simulink model "single_phase_inverter"  (R2026a)
settings: Solver=ode23tb  StopTime=param.sim.simlength  FixedStep=tc  MaxStep=param.glb_time.tc
values from neighbouring files (symbols this model uses):
  param = add_template_extras(param, options)    [init_model.m]
libraries: fl_lib x45, nesl_utility x24, single_phase_transformer_lib x3, phase_shift_filter x2, phase_shift_filter_ccaller x2, three_phase_voltage_with_frt_emulator x1, power_meter_iec x1, single_phase_transformer x1, three_phase_diode_rectifier x1, three_phase_diode_rectifier_with_thermal_model x1, full_bridge_ideal_switch x1, full_bridge_mosfet_based_with_thermal_model x1
(part 1 of 4)
settings Model: SimulationMode=accelerator  Creator=LTNBDA  LastModifiedBy=d.bagnara
settings SolverCC: ZeroCrossControl=DisableAll  ZeroCrossAlgorithm=Adaptive  SolverResetMethod=Robust
settings DataIOCC: MaxDataPoints=1  SignalLoggingSaveFormat=ModelDataLogs
settings OptimizationCC: InitFltsAndDblsToZero=on  EfficientMapNaN2IntZero=off
settings DebuggingCC: SaveWithParameterizedLinksMsg=none  SignalResolutionControl=TryResolveAllWithWarning  IgnoredZcDiagnostic=none  MultiTaskDSMMsg=warning  MultiTaskCondExecSysMsg=none  MultiTaskRateTransMsg=warning
settings HardwareCC: ProdBitPerLong=64.0  ProdHWDeviceType=Generic->64-bit Embedded Processor (LP64)  TargetBitPerPointer=64.0  TargetBitPerSizeT=64.0  TargetBitPerPtrDiffT=64.0  TargetLongLongMode=on  TargetIntDivRoundTo=Zero  TargetEndianess=LittleEndian  TargetWordSize=64.0  TargetHWDeviceType=MATLAB Host  ProdEqTarget=off
settings SFSimCC: SimCustomHeaderCode=|
  | #include "phase_shift_flt_simulink.h"
  | #include "sv_pwm.h"
  | #include "rpi.h"
  | #include "rpi_simulink.h"
  | #include "first_harmonic_tracker.h"
  | #include "dqvector_pi.h"
  | #include "dqvector_pi_simulink.h"
  | #include "sv_pwm_simulink.h"
  | #include "dqpll_grid.h"
  | #include "first_harmonic_tracker_simulink.h"
  | #include "dqpll_grid_simulink.h"
  | #include "phase_shift_flt.h"
  | #include "math_f.h"
  | #include "linear_double_integrator_observer_simulink.h"
  | #include "linear_double_integrator_observer.h"
  | #include "sogi_flt_simulink.h"
  | #include "sogi_flt.h"
settings SFSimCC: SimUserSources=|
  | "rpi.c"
  | "rpi_simulink.c"
  | "dqvector_pi_simulink.c"
  | "dqvector_pi.c"
  | "sv_pwm_simulink.c"
  | "sv_pwm.c"
  | "first_harmonic_tracker_simulink.c"
  | "first_harmonic_tracker.c"
  | "dqpll_grid_simulink.c"
  | "dqpll_grid.c"
  | "phase_shift_flt_simulink.c"
  | "phase_shift_flt.c"
  | "linear_double_integrator_observer_simulink.c"
  | "linear_double_integrator_observer.c"
  | "sogi_flt_simulink.c"
  | "sogi_flt.c"
settings SFSimCC: SimUserIncludeDirs=|
  | include
  | src
settings CodeAppCC: MaxIdLength=128.0
settings GRTTargetCC: CombineOutputUpdateFcns=off  GRTInterface=on
settings SimscapeCC: SimscapeNormalizeSystem=off  SimscapeNominalValues="[{\"value\":\"1\",\"unit\":\"A\"},{\"value\":\"1\",\"unit\":\"bar\"},{\"value\":\"1\",\"unit\":\"cm^2\"},{\"value\":\"1\",\"unit\":\"cm^3/s\"},{\"value\":\"1\",\"unit\":\"kJ/kg\"},{\"value\":\"1\",\"unit\":\"kW\"},{\"value\":\"1\",\"unit\":\"l\"},{\"value\":\"1\",\"unit\":\"N\"},{\"value\":\"1\",\"unit\":\"N*m\"},{\"value\":\"1\",\"unit\":\"V\"}]"  SimscapeLogType=none  SimscapeLogDataHistory=5000.0

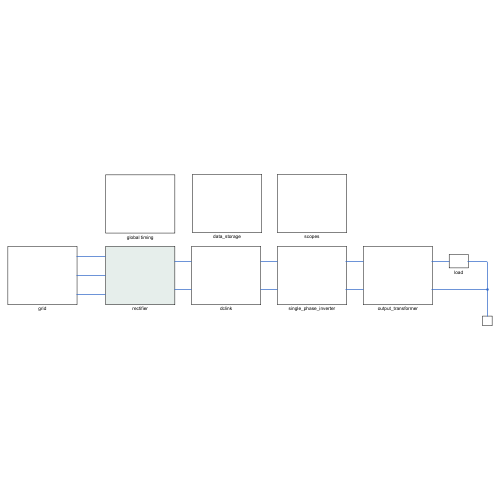
[thumbnail: Simulink's stored preview of the top-level diagram]
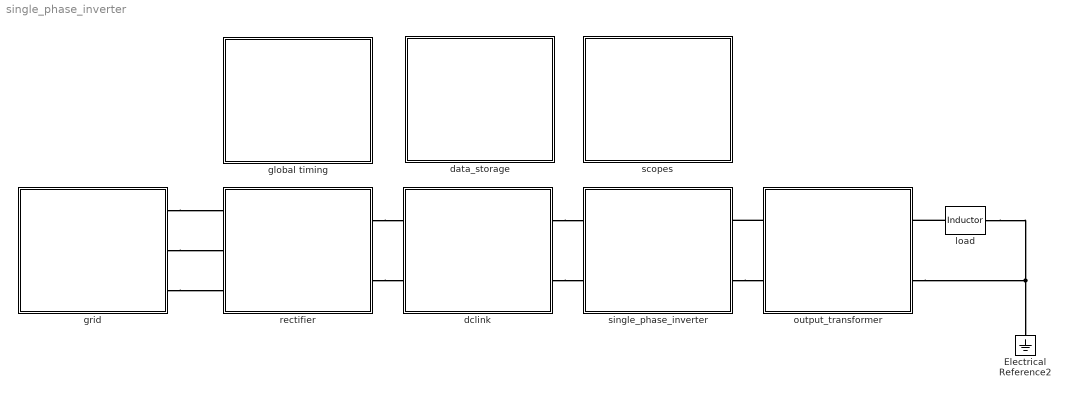
== system single_phase_inverter ==
  Electrical Reference2 : fl_lib/Electrical/Electrical Elements/Electrical Reference
  data_storage : Subsystem
  dclink : Subsystem
  global timing : Subsystem
  grid : Subsystem
  load : fl_lib/Electrical/Electrical Elements/Inductor  l=param.trafo_load.lload H  r=param.trafo_load.rload Ohm  g=1e-9 1/Ohm  i_specify=off  i_priority=None  i=0 A  i_nominal_specify=off  i_nominal_value=1  i_nominal_unit=A  v_specify=off  v_priority=None  v=0 V  v_nominal_specify=off  v_nominal_value=1  v_nominal_unit=V  i_L_specify=off  i_L_priority=High  i_L=0 A  i_L_nominal_specify=off  i_L_nominal_value=1  i_L_nominal_unit=A
  output_transformer : Subsystem
  rectifier : Subsystem
  scopes : Subsystem
  single_phase_inverter : Subsystem
  connections:
  dclink/RConn2 -- single_phase_inverter/LConn2
  dclink/RConn1 -- single_phase_inverter/LConn1
  rectifier/RConn1 -- dclink/LConn1
  rectifier/RConn2 -- dclink/LConn2
  output_transformer/LConn1 -- single_phase_inverter/RConn1
  single_phase_inverter/RConn2 -- output_transformer/LConn2
  output_transformer/RConn2 -- load/RConn1 -- Electrical Reference2/LConn1
  load/LConn1 -- output_transformer/RConn1
  grid/RConn3 -- rectifier/LConn3
  grid/RConn2 -- rectifier/LConn2
  grid/RConn1 -- rectifier/LConn1

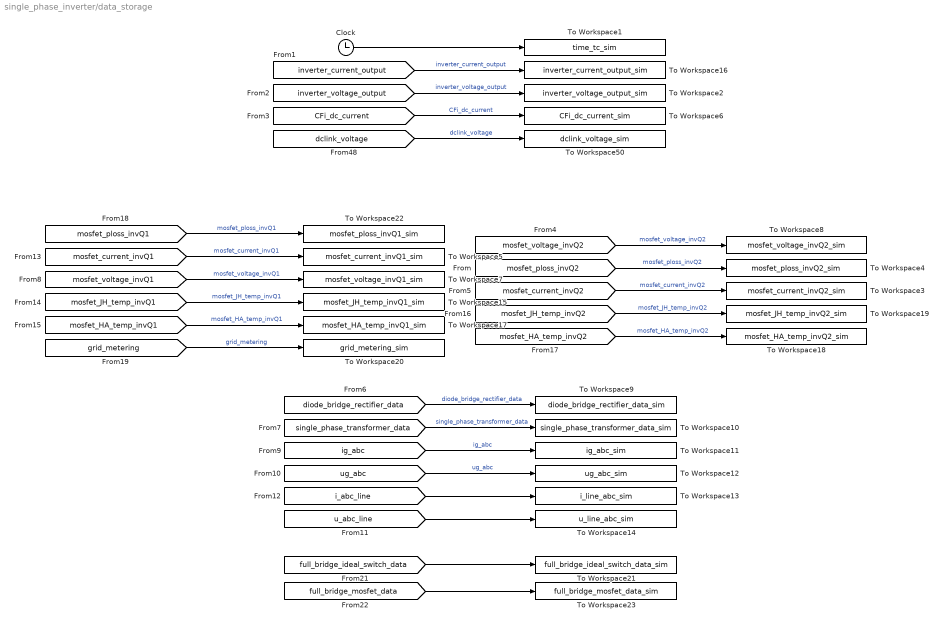
== system single_phase_inverter/data_storage ==
  Clock : Clock
  To Workspace1 : ToWorkspace  VariableName=time_tc_sim  SampleTime=param.glb_time.tc
      settings: MaxDataPoints=param.glb_time.Nc  Decimation=param.glb_time.decimation_tc
  To Workspace10 : ToWorkspace  VariableName=single_phase_transformer_data_sim  SampleTime=param.glb_time.tc
      settings: MaxDataPoints=param.glb_time.Nc  Decimation=param.glb_time.decimation_tc
  To Workspace11 : ToWorkspace  VariableName=ig_abc_sim  SampleTime=param.glb_time.tc
      settings: MaxDataPoints=param.glb_time.Nc  Decimation=param.glb_time.decimation_tc
  To Workspace12 : ToWorkspace  VariableName=ug_abc_sim  SampleTime=param.glb_time.tc
      settings: MaxDataPoints=param.glb_time.Nc  Decimation=param.glb_time.decimation_tc
  To Workspace13 : ToWorkspace  VariableName=i_line_abc_sim  SampleTime=param.glb_time.tc
      settings: MaxDataPoints=param.glb_time.Nc  Decimation=param.glb_time.decimation_tc
  To Workspace14 : ToWorkspace  VariableName=u_line_abc_sim  SampleTime=param.glb_time.tc
      settings: MaxDataPoints=param.glb_time.Nc  Decimation=param.glb_time.decimation_tc
  To Workspace15 : ToWorkspace  VariableName=mosfet_JH_temp_invQ1_sim  SampleTime=param.glb_time.tc
      settings: MaxDataPoints=param.glb_time.Nc  Decimation=param.glb_time.decimation_tc
  To Workspace16 : ToWorkspace  VariableName=inverter_current_output_sim  SampleTime=param.glb_time.tc
      settings: MaxDataPoints=param.glb_time.Nc  Decimation=param.glb_time.decimation_tc
  To Workspace17 : ToWorkspace  VariableName=mosfet_HA_temp_invQ1_sim  SampleTime=param.glb_time.tc
      settings: MaxDataPoints=param.glb_time.Nc  Decimation=param.glb_time.decimation_tc
  To Workspace18 : ToWorkspace  VariableName=mosfet_HA_temp_invQ2_sim  SampleTime=param.glb_time.tc
      settings: MaxDataPoints=param.glb_time.Nc  Decimation=param.glb_time.decimation_tc
  To Workspace19 : ToWorkspace  VariableName=mosfet_JH_temp_invQ2_sim  SampleTime=param.glb_time.tc
      settings: MaxDataPoints=param.glb_time.Nc  Decimation=param.glb_time.decimation_tc
  To Workspace2 : ToWorkspace  VariableName=inverter_voltage_output_sim  SampleTime=param.glb_time.tc
      settings: MaxDataPoints=param.glb_time.Nc  Decimation=param.glb_time.decimation_tc
  To Workspace20 : ToWorkspace  VariableName=grid_metering_sim  SampleTime=param.glb_time.tc
      settings: MaxDataPoints=param.glb_time.Nc  Decimation=param.glb_time.decimation_tc
  To Workspace21 : ToWorkspace  VariableName=full_bridge_ideal_switch_data_sim  SampleTime=param.glb_time.tc
      settings: MaxDataPoints=param.glb_time.Nc  Decimation=param.glb_time.decimation_tc
  To Workspace22 : ToWorkspace  VariableName=mosfet_ploss_invQ1_sim  SampleTime=param.glb_time.tc
      settings: MaxDataPoints=param.glb_time.Nc  Decimation=param.glb_time.decimation_tc
  To Workspace23 : ToWorkspace  VariableName=full_bridge_mosfet_data_sim  SampleTime=param.glb_time.tc
      settings: MaxDataPoints=param.glb_time.Nc  Decimation=param.glb_time.decimation_tc
  To Workspace3 : ToWorkspace  VariableName=mosfet_current_invQ2_sim  SampleTime=param.glb_time.tc
      settings: MaxDataPoints=param.glb_time.Nc  Decimation=param.glb_time.decimation_tc
  To Workspace4 : ToWorkspace  VariableName=mosfet_ploss_invQ2_sim  SampleTime=param.glb_time.tc
      settings: MaxDataPoints=param.glb_time.Nc  Decimation=param.glb_time.decimation_tc
  To Workspace5 : ToWorkspace  VariableName=mosfet_current_invQ1_sim  SampleTime=param.glb_time.tc
      settings: MaxDataPoints=param.glb_time.Nc  Decimation=param.glb_time.decimation_tc
  To Workspace50 : ToWorkspace  VariableName=dclink_voltage_sim  SampleTime=param.glb_time.tc
      settings: MaxDataPoints=param.glb_time.Nc  Decimation=param.glb_time.decimation_tc
  To Workspace6 : ToWorkspace  VariableName=CFi_dc_current_sim  SampleTime=param.glb_time.tc
      settings: MaxDataPoints=param.glb_time.Nc  Decimation=param.glb_time.decimation_tc
  To Workspace7 : ToWorkspace  VariableName=mosfet_voltage_invQ1_sim  SampleTime=param.glb_time.tc
      settings: MaxDataPoints=param.glb_time.Nc  Decimation=param.glb_time.decimation_tc
  To Workspace8 : ToWorkspace  VariableName=mosfet_voltage_invQ2_sim  SampleTime=param.glb_time.tc
      settings: MaxDataPoints=param.glb_time.Nc  Decimation=param.glb_time.decimation_tc
  To Workspace9 : ToWorkspace  VariableName=diode_bridge_rectifier_data_sim  SampleTime=param.glb_time.tc
      settings: MaxDataPoints=param.glb_time.Nc  Decimation=param.glb_time.decimation_tc
  wires:
  Clock/1 -> To Workspace1/1
  [inverter_current_output] -> To Workspace16/1  "inverter_current_output"
  [inverter_voltage_output] -> To Workspace2/1  "inverter_voltage_output"
  [CFi_dc_current] -> To Workspace6/1  "CFi_dc_current"
  [mosfet_ploss_invQ1] -> To Workspace22/1  "mosfet_ploss_invQ1"
  [dclink_voltage] -> To Workspace50/1  "dclink_voltage"
  [mosfet_current_invQ1] -> To Workspace5/1  "mosfet_current_invQ1"
  [mosfet_current_invQ2] -> To Workspace3/1  "mosfet_current_invQ2"
  [mosfet_ploss_invQ2] -> To Workspace4/1  "mosfet_ploss_invQ2"
  [mosfet_voltage_invQ1] -> To Workspace7/1  "mosfet_voltage_invQ1"
  [mosfet_voltage_invQ2] -> To Workspace8/1  "mosfet_voltage_invQ2"
  [diode_bridge_rectifier_data] -> To Workspace9/1  "diode_bridge_rectifier_data"
  [single_phase_transformer_data] -> To Workspace10/1  "single_phase_transformer_data"
  [ig_abc] -> To Workspace11/1  "ig_abc"
  [ug_abc] -> To Workspace12/1  "ug_abc"
  [i_abc_line] -> To Workspace13/1
  [u_abc_line] -> To Workspace14/1
  [mosfet_JH_temp_invQ1] -> To Workspace15/1  "mosfet_JH_temp_invQ1"
  [mosfet_HA_temp_invQ1] -> To Workspace17/1  "mosfet_HA_temp_invQ1"
  [mosfet_JH_temp_invQ2] -> To Workspace19/1  "mosfet_JH_temp_invQ2"
  [mosfet_HA_temp_invQ2] -> To Workspace18/1  "mosfet_HA_temp_invQ2"
  [grid_metering] -> To Workspace20/1  "grid_metering"
  [full_bridge_mosfet_data] -> To Workspace23/1
  [full_bridge_ideal_switch_data] -> To Workspace21/1

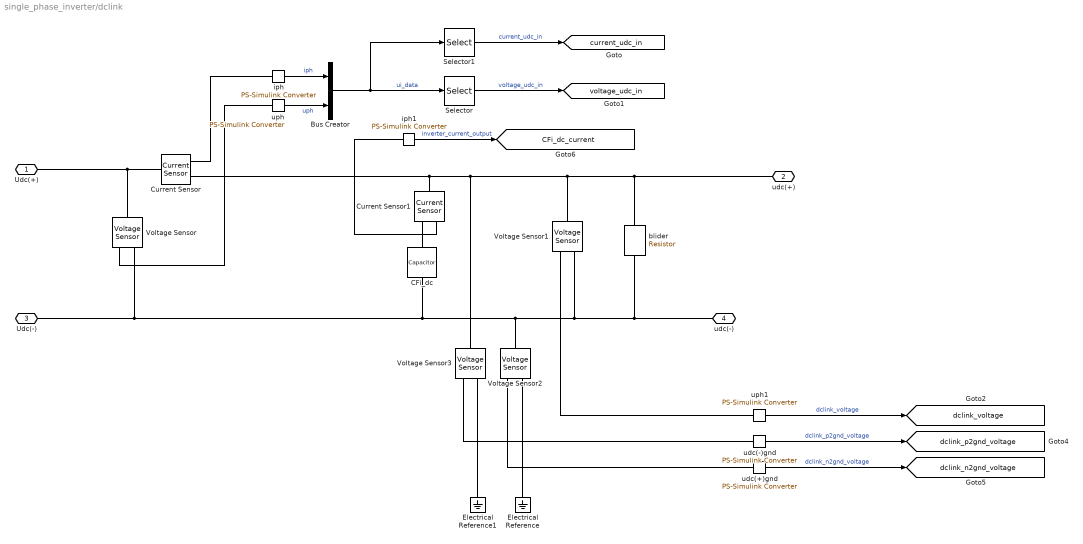
== system single_phase_inverter/dclink ==
  Bus Creator : BusCreator  Inputs=2
  CFi_dc : fl_lib/Electrical/Electrical Elements/Capacitor  c=param.spinv.hw.CFi F  r=param.spinv.hw.RCFi Ohm  g=0 1/Ohm  i_specify=off  i_priority=None  i=0 A  i_nominal_specify=off  i_nominal_value=1  i_nominal_unit=A  v_specify=off  v_priority=None  v=0 V  v_nominal_specify=off  v_nominal_value=1  v_nominal_unit=V  vc_specify=off  vc_priority=High  vc=0 V  vc_nominal_specify=off  vc_nominal_value=1  vc_nominal_unit=V
  Current Sensor : fl_lib/Electrical/Electrical Sensors/Current Sensor
  Current Sensor1 : fl_lib/Electrical/Electrical Sensors/Current Sensor
  Electrical Reference : fl_lib/Electrical/Electrical Elements/Electrical Reference
  Electrical Reference1 : fl_lib/Electrical/Electrical Elements/Electrical Reference
  Selector : Selector  InputPortWidth=2  IndexOptions=Index vector (dialog)  Indices=2  OutputSizes=1
  Selector1 : Selector  InputPortWidth=2  IndexOptions=Index vector (dialog)  Indices=1  OutputSizes=1
  Voltage Sensor{,1..3} (4 alike) : fl_lib/Electrical/Electrical Sensors/Voltage Sensor
  blider : fl_lib/Electrical/Electrical Elements/Resistor  R=1200 Ohm  i_specify=off  i_priority=None  i=0 A  i_nominal_specify=off  i_nominal_value=1  i_nominal_unit=A  v_specify=off  v_priority=None  v=0 V  v_nominal_specify=off  v_nominal_value=1  v_nominal_unit=V
  iph : nesl_utility/PS-Simulink Converter  PhysicalDomain=network_engine_domain  SubClassName=ps_output  LeftPortType=input  RightPortType=output  PseudoPeriodic=off  Frequencies=[]  VectorFormat=1-D array  Unit=A  AffineConversion=off
  iph1 : nesl_utility/PS-Simulink Converter  PhysicalDomain=network_engine_domain  SubClassName=ps_output  LeftPortType=input  RightPortType=output  PseudoPeriodic=off  Frequencies=[]  VectorFormat=1-D array  Unit=A  AffineConversion=off
  udc(+)gnd : nesl_utility/PS-Simulink Converter  PhysicalDomain=network_engine_domain  SubClassName=ps_output  LeftPortType=input  RightPortType=output  PseudoPeriodic=off  Frequencies=[]  VectorFormat=1-D array  Unit=V  AffineConversion=off
  udc(-)gnd : nesl_utility/PS-Simulink Converter  PhysicalDomain=network_engine_domain  SubClassName=ps_output  LeftPortType=input  RightPortType=output  PseudoPeriodic=off  Frequencies=[]  VectorFormat=1-D array  Unit=V  AffineConversion=off
  uph : nesl_utility/PS-Simulink Converter  PhysicalDomain=network_engine_domain  SubClassName=ps_output  LeftPortType=input  RightPortType=output  PseudoPeriodic=off  Frequencies=[]  VectorFormat=1-D array  Unit=V  AffineConversion=off
  uph1 : nesl_utility/PS-Simulink Converter  PhysicalDomain=network_engine_domain  SubClassName=ps_output  LeftPortType=input  RightPortType=output  PseudoPeriodic=off  Frequencies=[]  VectorFormat=1-D array  Unit=V  AffineConversion=off
  Udc(+) : PMIOPort  Side=Left
  udc(+) : PMIOPort  Port=2  Side=Right
  Udc(-) : PMIOPort  Port=3  Side=Left
  udc(-) : PMIOPort  Port=4  Side=Right
  tag scope: CFi_dc_current=global, current_udc_in=global, dclink_n2gnd_voltage=global, dclink_p2gnd_voltage=global, dclink_voltage=global, voltage_udc_in=global
  wires:
  Bus Creator/1 -> Selector/1, Selector1/1  "ui_data"
  iph/1 -> Bus Creator/1  "iph"
  uph/1 -> Bus Creator/2  "uph"
  Selector1/1 -> [current_udc_in]  "current_udc_in"
  Selector/1 -> [voltage_udc_in]  "voltage_udc_in"
  iph1/1 -> [CFi_dc_current]  "inverter_current_output"
  udc(+)gnd/1 -> [dclink_n2gnd_voltage]  "dclink_n2gnd_voltage"
  uph1/1 -> [dclink_voltage]  "dclink_voltage"
  udc(-)gnd/1 -> [dclink_p2gnd_voltage]  "dclink_p2gnd_voltage"
  connections:
  iph/LConn1 -- Current Sensor/RConn1
  Voltage Sensor/LConn1 -- Current Sensor/LConn1 -- Udc(+)/RConn1
  Voltage Sensor/RConn1 -- uph/LConn1
  CFi_dc/RConn1 -- Voltage Sensor1/RConn2 -- udc(-)/RConn1 -- blider/RConn1 -- Voltage Sensor2/LConn1 -- Voltage Sensor/RConn2 -- Udc(-)/RConn1
  udc(+)/RConn1 -- blider/LConn1 -- Voltage Sensor1/LConn1 -- Voltage Sensor3/LConn1 -- Current Sensor/RConn2 -- Current Sensor1/LConn1
  Current Sensor1/RConn2 -- CFi_dc/LConn1
  Electrical Reference1/LConn1 -- Voltage Sensor3/RConn2
  udc(-)gnd/LConn1 -- Voltage Sensor3/RConn1
  Voltage Sensor2/RConn1 -- udc(+)gnd/LConn1
  Electrical Reference/LConn1 -- Voltage Sensor2/RConn2
  Voltage Sensor1/RConn1 -- uph1/LConn1
  Current Sensor1/RConn1 -- iph1/LConn1

== system single_phase_inverter/global timing ==
  Unit Delay : UnitDelay  SampleTime=param.glb_time.tc
  time_afe1 : Subsystem  mask{k=1}
      mask prompts: k "Time Gain"
      mask Display:
      | disp('time-gen');
      | port_label('input', 1, 'crt');
      | port_label('output', 1, 'tout');
  time_afe3 : Subsystem  mask{k=1}
      mask prompts: k "Time Gain"
      mask Display:
      | disp('time-gen');
      | port_label('output', 1, 'tout');
  tag scope: master_time=global, time_inv_module_1=global
  wires:
  time_afe1/1(Out1) -> [time_inv_module_1]
  time_afe3/1(Out1) -> [master_time]
  [local_time_corr_llc_mod1] -> Unit Delay/1
  Unit Delay/1 -> time_afe1/1(correction_time)

== system single_phase_inverter/grid ==
  Bus Selector : BusSelector  OutputSignals=Q1p,Q1n,P1n,P1p,U1n,U1p,i_act_1n,i_react_1n,i_act_1p,i_react_1p
  To Workspace1 : ToWorkspace  VariableName=i_react_1n  SampleTime=param.glb_time.ts_afe
      settings: MaxDataPoints=param.glb_time.Ns_afe
  To Workspace2 : ToWorkspace  VariableName=i_react_1p  SampleTime=param.glb_time.ts_afe
      settings: MaxDataPoints=param.glb_time.Ns_afe
  To Workspace3 : ToWorkspace  VariableName=i_act_1n  SampleTime=param.glb_time.ts_afe
      settings: MaxDataPoints=param.glb_time.Ns_afe
  To Workspace4 : ToWorkspace  VariableName=i_act_1p  SampleTime=param.glb_time.ts_afe
      settings: MaxDataPoints=param.glb_time.Ns_afe
  To Workspace5 : ToWorkspace  VariableName=u1p  SampleTime=param.glb_time.ts_afe
      settings: MaxDataPoints=param.glb_time.Ns_afe
  To Workspace6 : ToWorkspace  VariableName=u1n  SampleTime=param.glb_time.ts_afe
      settings: MaxDataPoints=param.glb_time.Ns_afe
  grid_emulator : Subsystem
  power meter iec : power_meter_iec/power meter iec  period=pi/param.grid.emu.omega_grid_nom  ts=param.glb_time.ts_afe  enable_time=0.025
  threephase_vi_measures : Subsystem
  ua : PMIOPort  Side=Right
  ub : PMIOPort  Port=2  Side=Right
  uc : PMIOPort  Port=3  Side=Right
  tag scope: P1n_global=global, P1p_global=global, Q1n_global=global, Q1p_global=global, grid_metering=global
  wires:
  [gamma_grid_emulator] -> power meter iec/1
  [ug_abc] -> power meter iec/2
  [ig_abc] -> power meter iec/3
  power meter iec/1 -> [grid_metering], Bus Selector/1
  Bus Selector/1 -> [Q1p_global]  "<Q1p>"
  Bus Selector/2 -> [Q1n_global]  "<Q1n>"
  Bus Selector/3 -> [P1n_global]  "<P1n>"
  Bus Selector/4 -> [P1p_global]  "<P1p>"
  Bus Selector/5 -> To Workspace6/1  "<U1n>"
  Bus Selector/6 -> To Workspace5/1  "<U1p>"
  Bus Selector/7 -> To Workspace3/1  "<i_act_1n>"
  Bus Selector/8 -> To Workspace1/1  "<i_react_1n>"
  Bus Selector/9 -> To Workspace4/1  "<i_act_1p>"
  Bus Selector/10 -> To Workspace2/1  "<i_react_1p>"
  [omega_grid_emulator] -> power meter iec/4
  connections:
  threephase_vi_measures/LConn3 -- grid_emulator/RConn3
  threephase_vi_measures/LConn1 -- grid_emulator/RConn1
  threephase_vi_measures/RConn2 -- ub/RConn1
  threephase_vi_measures/LConn2 -- grid_emulator/RConn2
  threephase_vi_measures/RConn1 -- ua/RConn1
  threephase_vi_measures/RConn3 -- uc/RConn1

== system single_phase_inverter/output_transformer ==
  single_phase_transformer : single_phase_transformer/single_phase_transformer  lm_trafo=param.trafo_load.output_transformer.Lm1  m1=param.trafo_load.output_transformer.n1  m2=param.trafo_load.output_transformer.n2  rd1_trafo=param.trafo_load.output_transformer.Rd1  rd2_trafo=0  ld1_trafo=2*param.trafo_load.output_transformer.Ld1  ld2_trafo=0  rfe_trafo=param.trafo_load.output_transformer.Rfe1  length_core=1  mu0=1.256637e-6  mur=1200
  single_phase_transformer - scope : Scope
      settings: ActiveDisplayYMinimum=-52667.127888169394  ActiveDisplayYMaximum=52594.361496045676  DataLoggingVariableName=ScopeData11
  u1(+) : PMIOPort  Side=Left
  u2(+) : PMIOPort  Port=2  Side=Right
  u1(-) : PMIOPort  Port=3  Side=Left
  u2(-) : PMIOPort  Port=4  Side=Right
  tag scope: single_phase_transformer_data=global
  wires:
  single_phase_transformer/1 -> [single_phase_transformer_data], single_phase_transformer - scope/1
  connections:
  single_phase_transformer/LConn2 -- u1(-)/RConn1
  single_phase_transformer/LConn1 -- u1(+)/RConn1
  single_phase_transformer/RConn1 -- u2(+)/RConn1
  single_phase_transformer/RConn2 -- u2(-)/RConn1

== system single_phase_inverter/rectifier ==
  H5_filter : Subsystem  Commented=on
  H7_filter : Subsystem  Commented=on
  three phase diode rectifier : three_phase_diode_rectifier/three phase diode rectifier  Commented=on  Vf_diode_rectifier=param.diode.rectifier.Vf  Rdon_diode_rectifier=param.diode.rectifier.Rdon  Csnubber=param.spinv.igbt.Csnubber  Rsnubber=param.spinv.igbt.Rsnubber
  three_phase_diode_rectifier_with_thermal_model : three_phase_diode_rectifier_with_thermal_model/three_phase_diode_rectifier_with_thermal_model  Vf_diode_rectifier=param.diode.rectifier.Vf  Rdon_diode_rectifier=param.diode.rectifier.Rdon  mass_heatsink_m=param.thermal.heatsink.no_weight  specific_heat_m=param.thermal.heatsink.cp  rth_diode_JH_m=param.spinv.igbt.Rth_diode_JH  rth_diode_HA_m=param.thermal.Rth_mosfet_HA  Csnubber=param.spinv.igbt.Csnubber  Rsnubber=param.spinv.igbt.Rsnubber
      link override diode_3/Goto2: GotoTag=diode3_JH_temperature
  us_a : PMIOPort  Side=Left
  us_b : PMIOPort  Port=2  Side=Left
  us_c : PMIOPort  Port=3  Side=Left
  Udc(+) : PMIOPort  Port=4  Side=Right
  Udc(-) : PMIOPort  Port=5  Side=Right
  tag scope: diode_bridge_rectifier_data=global
  wires:
  three_phase_diode_rectifier_with_thermal_model/1 -> [diode_bridge_rectifier_data]
  connections:
  Udc(+)/RConn1 -- three_phase_diode_rectifier_with_thermal_model/RConn1 -- three phase diode rectifier/RConn1
  Udc(-)/RConn1 -- three_phase_diode_rectifier_with_thermal_model/RConn2 -- three phase diode rectifier/RConn2
  H5_filter/LConn1 -- us_a/RConn1 -- three_phase_diode_rectifier_with_thermal_model/LConn1 -- three phase diode rectifier/LConn1 -- H7_filter/LConn1
  H5_filter/LConn2 -- us_b/RConn1 -- three phase diode rectifier/LConn2 -- three_phase_diode_rectifier_with_thermal_model/LConn2 -- H7_filter/LConn2
  H5_filter/LConn3 -- us_c/RConn1 -- three_phase_diode_rectifier_with_thermal_model/LConn3 -- three phase diode rectifier/LConn3 -- H7_filter/LConn3

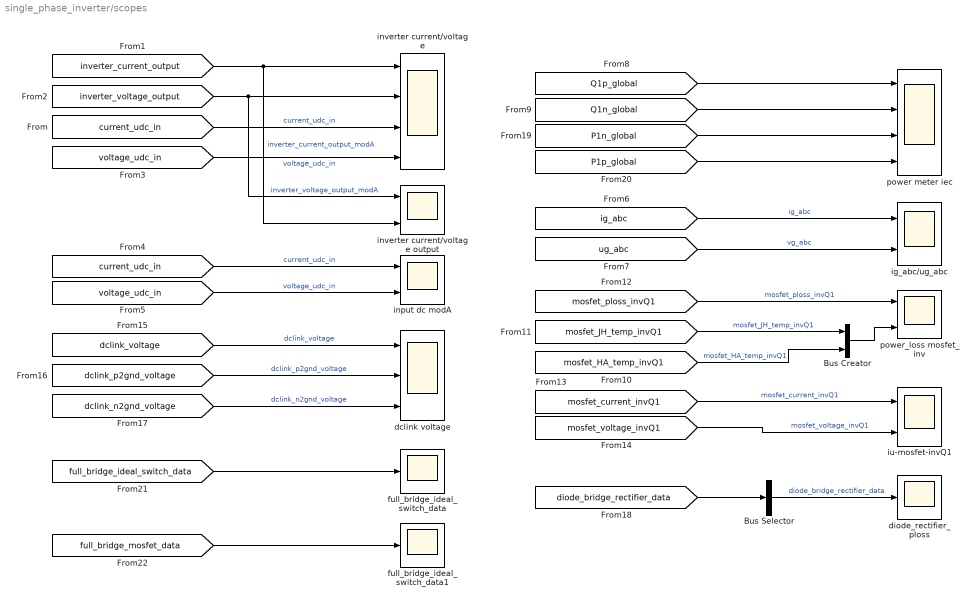
== system single_phase_inverter/scopes ==
  Bus Creator : BusCreator  Inputs=2
  Bus Selector : BusSelector  OutputSignals=diode1_ploss,diode6_ploss,diode5_ploss,diode4_ploss,diode3_ploss,diode2_ploss  OutputAsBus=on
  dclink voltage : Scope  NumInputPorts=3
      settings: SampleTime=param.glb_time.tc  ActiveDisplayString=3  ActiveDisplayYMinimum=-363.18697781386322  ActiveDisplayYMaximum=-188.17161920145585  DataLoggingVariableName=ScopeData9
  diode_rectifier_ploss : Scope
      settings: ActiveDisplayYMinimum=-388.41488046396341  ActiveDisplayYMaximum=3494.091610714474  DataLoggingVariableName=ScopeData13
  full_bridge_ideal_switch_data : Scope
      settings: ActiveDisplayYMinimum=-388.41488046396341  ActiveDisplayYMaximum=3494.091610714474  DataLoggingVariableName=ScopeData17
  full_bridge_ideal_switch_data1 : Scope
      settings: ActiveDisplayYMinimum=-388.41488046396341  ActiveDisplayYMaximum=3494.091610714474  DataLoggingVariableName=ScopeData18
  ig_abc/ug_abc : Scope  NumInputPorts=2
      settings: SampleTime=param.glb_time.tc  ActiveDisplayYMinimum=-781.78189031693421  ActiveDisplayYMaximum=781.86071704862093  DataLoggingVariableName=ScopeData5
  input dc modA : Scope  NumInputPorts=2
      settings: SampleTime=param.glb_time.tc  ActiveDisplayYMinimum=-264.41735822415785  ActiveDisplayYMaximum=1802.2815575209611  DataLoggingVariableName=ScopeData4
  inverter current/voltage : Scope  NumInputPorts=4
      settings: ActiveDisplayString=3  ActiveDisplayYMinimum=-93.6274374097306  ActiveDisplayYMaximum=842.6107714271742
  inverter current/voltage output : Scope  NumInputPorts=2
      settings: ActiveDisplayYMinimum=-719.5057944888872  ActiveDisplayYMaximum=719.52818794442339
  iu-mosfet-invQ1 : Scope  NumInputPorts=2
      settings: SampleTime=param.glb_time.tc  ActiveDisplayYMinimum=-1884.5917198054758  ActiveDisplayYMaximum=2532.7760155502147  DataLoggingVariableName=ScopeData7
  power meter iec : Scope  NumInputPorts=4
      settings: ActiveDisplayString=3  ActiveDisplayYMinimum=-178.52926094214885  ActiveDisplayYMaximum=1606.7629741781627  DataLoggingVariableName=ScopeData16
  power_loss mosfet_inv : Scope  NumInputPorts=2
      settings: SampleTime=param.glb_time.tc  ActiveDisplayYMinimum=-70.3597503046535  ActiveDisplayYMaximum=633.23512274412  DataLoggingVariableName=ScopeData6
  wires:
  [current_udc_in] -> inverter current/voltage/3  "current_udc_in"
  [inverter_voltage_output] -> inverter current/voltage output/1, inverter current/voltage/2  "inverter_voltage_output_modA"
  [inverter_current_output] -> inverter current/voltage output/2, inverter current/voltage/1  "inverter_current_output_modA"
  [voltage_udc_in] -> inverter current/voltage/4  "voltage_udc_in"
  [current_udc_in] -> input dc modA/1  "current_udc_in"
  [voltage_udc_in] -> input dc modA/2  "voltage_udc_in"
  [ug_abc] -> ig_abc/ug_abc/2  "vg_abc"
  [ig_abc] -> ig_abc/ug_abc/1  "ig_abc"
  [mosfet_ploss_invQ1] -> power_loss mosfet_inv/1  "mosfet_ploss_invQ1"
  [mosfet_JH_temp_invQ1] -> Bus Creator/1  "mosfet_JH_temp_invQ1"
  [mosfet_HA_temp_invQ1] -> Bus Creator/2  "mosfet_HA_temp_invQ1"
  Bus Creator/1 -> power_loss mosfet_inv/2
  [mosfet_current_invQ1] -> iu-mosfet-invQ1/1  "mosfet_current_invQ1"
  [mosfet_voltage_invQ1] -> iu-mosfet-invQ1/2  "mosfet_voltage_invQ1"
  [dclink_voltage] -> dclink voltage/1  "dclink_voltage"
  [dclink_p2gnd_voltage] -> dclink voltage/2  "dclink_p2gnd_voltage"
  [dclink_n2gnd_voltage] -> dclink voltage/3  "dclink_n2gnd_voltage"
  [diode_bridge_rectifier_data] -> Bus Selector/1
  Bus Selector/1 -> diode_rectifier_ploss/1  "diode_bridge_rectifier_data"
  [Q1p_global] -> power meter iec/1
  [Q1n_global] -> power meter iec/2
  [P1n_global] -> power meter iec/3
  [P1p_global] -> power meter iec/4
  [full_bridge_ideal_switch_data] -> full_bridge_ideal_switch_data/1
  [full_bridge_mosfet_data] -> full_bridge_ideal_switch_data1/1

== system single_phase_inverter/single_phase_inverter ==
  Current Sensor : fl_lib/Electrical/Electrical Sensors/Current Sensor
  Voltage Sensor1 : fl_lib/Electrical/Electrical Sensors/Voltage Sensor
  iph : nesl_utility/PS-Simulink Converter  PhysicalDomain=network_engine_domain  SubClassName=ps_output  LeftPortType=input  RightPortType=output  PseudoPeriodic=off  Frequencies=[]  VectorFormat=1-D array  Unit=A  AffineConversion=off
  single phase inverter : Subsystem
      settings: PortSchema="{\"entries\":[{\"content\":{\"sides\":[{\"content\":{\"connectorIds\":[\"LConn1\",\"LConn2\"]},\"type\":\"ConnectorPlacement.EquallySpacedRectSide\",\"uuid\":\"4fcf4fea-d38f-431b-8a91-be3ce9782faf\"},{\"content\":{\"connectorIds\":[\"RConn1\",\"RConn2\"],\"side\":\"RIGHT\"},\"type\":\"ConnectorPlacement.EquallySpacedRectSide\",\"uuid\":\"0aa56277-92e9-4e3b-84c7-43398254a4d8\"},{\"content\":{\"connectorIds\":[\"In1\"],\"side\":\"TOP\"},\"type\":\"ConnectorPlacement.EquallySpacedRectSide\",\"uuid\":\"5cd150dc-bcaf-4cd7-b2a8-3db203726730\"}]},\"type\":\"ConnectorPlacement.EquallySpacedConnector\",\"uuid\":\"bf8194c4-c327-4d40-bea4-f1e7617f80b4\"}],\"packageUris\":[\"http://schema.mathworks.com/mf0/Connector/R2020b\"],\"version\":\"1.0\"}"
  single phase inverter control : Subsystem
  uph1 : nesl_utility/PS-Simulink Converter  PhysicalDomain=network_engine_domain  SubClassName=ps_output  LeftPortType=input  RightPortType=output  PseudoPeriodic=off  Frequencies=[]  VectorFormat=1-D array  Unit=V  AffineConversion=off
  uac(+) : PMIOPort  Side=Right
  uac(-) : PMIOPort  Port=2  Side=Right
  udc(+) : PMIOPort  Port=3  Side=Left
  udc(-) : PMIOPort  Port=4  Side=Left
  tag scope: inverter_current_output=global, inverter_voltage_output=global
  wires:
  single phase inverter control/1(gate_cmds) -> single phase inverter/1(gate_commands)
  iph/1 -> [inverter_current_output]  "inverter_current_output"
  uph1/1 -> [inverter_voltage_output]  "inverter_voltage_output"
  connections:
  Current Sensor/LConn1 -- single phase inverter/LConn1
  uac(-)/RConn1 -- single phase inverter/LConn2 -- Voltage Sensor1/RConn2
  Voltage Sensor1/RConn1 -- uph1/LConn1
  iph/LConn1 -- Current Sensor/RConn1
  uac(+)/RConn1 -- Current Sensor/RConn2 -- Voltage Sensor1/LConn1
  udc(+)/RConn1 -- single phase inverter/RConn1
  udc(-)/RConn1 -- single phase inverter/RConn2

== system single_phase_inverter/global timing/time_afe1 ==
  correction_time : Inport
  Constant : Constant
  Gain : Gain  Gain=k
  Product : Product
  Sum : Sum  Inputs=|++
  time_1 : Clock
  Out1 : Outport
  wires:
  time_1/1 -> Gain/1
  Gain/1 -> Product/1
  Product/1 -> Out1/1
  correction_time/1 -> Sum/1
  Sum/1 -> Product/2
  Constant/1 -> Sum/2

== system single_phase_inverter/global timing/time_afe3 ==
  Gain : Gain  Gain=k
  time_1 : Clock
  Out1 : Outport
  wires:
  Gain/1 -> Out1/1
  time_1/1 -> Gain/1

== system single_phase_inverter/grid/grid_emulator ==
  3ph_Dyg : Subsystem
  Bus Selector : BusSelector  OutputSignals=ua_grid_emu,ub_grid_emu,uc_grid_emu
  Bus Selector1 : BusSelector  OutputSignals=gamma_grid_emulator,omega_grid_emulator
  Controlled Voltage Source : fl_lib/Electrical/Electrical Sources/Controlled Voltage Source
  Controlled Voltage Source1 : fl_lib/Electrical/Electrical Sources/Controlled Voltage Source
  Controlled Voltage Source2 : fl_lib/Electrical/Electrical Sources/Controlled Voltage Source
  Electrical Reference : fl_lib/Electrical/Electrical Elements/Electrical Reference
  Simulink-PS Converter : nesl_utility/Simulink-PS Converter  PhysicalDomain=network_engine_domain  SubClassName=ps_input  LeftPortType=input  RightPortType=output  PseudoPeriodic=off  Frequencies=[]  NoiseDistribution=none  NoiseParameters=[]  Unit=V  AffineConversion=on  FilteringAndDerivatives=provide  SimscapeFilterOrder=1  InputFilterTimeConstant=0.001  UdotUserProvided=0
  Simulink-PS Converter1 : nesl_utility/Simulink-PS Converter  PhysicalDomain=network_engine_domain  SubClassName=ps_input  LeftPortType=input  RightPortType=output  PseudoPeriodic=off  Frequencies=[]  NoiseDistribution=none  NoiseParameters=[]  Unit=V  AffineConversion=on  FilteringAndDerivatives=provide  SimscapeFilterOrder=1  InputFilterTimeConstant=0.001  UdotUserProvided=0
  Simulink-PS Converter2 : nesl_utility/Simulink-PS Converter  PhysicalDomain=network_engine_domain  SubClassName=ps_input  LeftPortType=input  RightPortType=output  PseudoPeriodic=off  Frequencies=[]  NoiseDistribution=none  NoiseParameters=[]  Unit=V  AffineConversion=on  FilteringAndDerivatives=provide  SimscapeFilterOrder=1  InputFilterTimeConstant=0.001  UdotUserProvided=0
  Solver Configuration : nesl_utility/Solver Configuration  PhysicalDomain=network_engine_domain  SubClassName=solver  LeftPortType=input  RightPortType=generic  Tones=[]  Harmonics=[]  SimulateNoise=off  Profile=off  UseLocalSampling=off  EnableSwitchedLinearOptims=on  FrequencyDomain=off  UseCCode=off  RelTol=0.001  AbsTol=0.001  MinStep=1e-09  ToWorkspace=off  RevertToSquareIcSolve=off  NumHomotopyIterations=100  PhasorMode=off  PhasorModeNumHarmonics=1  ConsistencySolver=NEWTON_FTOL  CanonicalOrdering=UNORDERED  OptimizeIntermediates=UNOPTIMIZED  IndexReductionMethod=DerivativeReplacement  DoDC=on  ResidualTolerance=1e-09  ConsistencyTolSource=GLOBAL  ConsistencyAbsTol=0.001  ConsistencyRelTol=0.001  ConsistencyTolFactor=0.001  UseLocalSolver=on  LocalSolverChoice=NE_BACKWARD_EULER_ADVANCER  ResolveIndetEquations=on  FunctionEvalNumThread=1  LocalSolverSampleTime=param.glb_time.tc  DoFixedCost=on  MaxNonlinIter=param.sim.nonlinear_iterations  MaxModeIter=2  ComputeImpulses=off  ImpulseIterations=2  LinearAlgebra=auto  LinearAlgebraNumThread=0  EquationFormulation=NE_TIME_EF  DelaysMemoryBudget=1024  AutomaticFiltering=on  FilteringTimeConstant=0.001  PartitionStorageMethod=AS_NEEDED  PartitionMemoryBudget=1024  PartitionMethod=ROBUST  MultibodyUseLocalSolver=off  MultibodyLocalSolverChoice=ODE1  MultibodyLocalSolverSampleTime=0.001
  three_phase_voltage_source_with_frt_emulator : three_phase_voltage_with_frt_emulator/three_phase_voltage_source_with_frt_emulator  nominal_frequency_m=param.grid.emu.fgrid_nom  nominal_voltage_m=param.grid.emu.us_primary_nom  Vemu_ref_norm_m=param.grid.emu.Vemu_ref_norm  vp_xi_pu_m=param.grid.emu.up_xi_pu_ref  vp_eta_pu_m=param.grid.emu.up_eta_pu_ref  vn_xi_pu_m=param.grid.emu.un_xi_pu_ref  vn_eta_pu_m=param.grid.emu.un_eta_pu_ref  Am=param.ctrl.filters.afe.SOF_50Hz.ss_c.A  Bm=param.ctrl.filters.afe.SOF_50Hz.ss_c.B  Cm=param.ctrl.filters.afe.SOF_50Hz.ss_c.C  enable_frt_1_m=param.frt.data.enable_frt_1  enable_frt_2_m=param.frt.data.enable_frt_2  start_time_LVRT_m=param.frt.data.start_time_LVRT  end_time_LVRT_m=param.frt.data.end_time_LVRT  deepPOSxi_m=param.frt.data.deepPOSxi  deepPOSeta_m=param.frt.data.deepPOSeta  deepNEGxi_m=param.frt.data.deepNEGxi  deepNEGeta_m=param.frt.data.deepNEGeta  Amplitude_U_m=param.frt.data.Amplitude_U  Amplitude_V_m=param.frt.data.Amplitude_V  Amplitude_W_m=param.frt.data.Amplitude_W  t_ramp_m=param.frt.data.t_ramp  Phase_shift_m=param.frt.data.Phase_shift
  threephase_vi_measures : Subsystem
  u1 : PMIOPort  Side=Right
  u2 : PMIOPort  Port=2  Side=Right
  u3 : PMIOPort  Port=3  Side=Right
  tag scope: gamma_grid_emulator=global, omega_grid_emulator=global
  wires:
  Bus Selector1/2 -> [omega_grid_emulator]  "<omega_grid_emulator>"
  Bus Selector1/1 -> [gamma_grid_emulator]  "<gamma_grid_emulator>"
  Bus Selector/2 -> Simulink-PS Converter1/1  "<ub_grid_emu>"
  Bus Selector/3 -> Simulink-PS Converter2/1  "<uc_grid_emu>"
  three_phase_voltage_source_with_frt_emulator/1 -> Bus Selector1/1, Bus Selector/1
  Bus Selector/1 -> Simulink-PS Converter/1  "<ua_grid_emu>"
  connections:
  Simulink-PS Converter/RConn1 -- Controlled Voltage Source/RConn1
  Simulink-PS Converter1/RConn1 -- Controlled Voltage Source1/RConn1
  Simulink-PS Converter2/RConn1 -- Controlled Voltage Source2/RConn1
  Controlled Voltage Source/RConn2 -- Controlled Voltage Source1/RConn2 -- Controlled Voltage Source2/RConn2 -- Electrical Reference/LConn1 -- Solver Configuration/RConn1
  3ph_Dyg/RConn1 -- u1/RConn1
  3ph_Dyg/RConn2 -- u2/RConn1
  3ph_Dyg/RConn3 -- u3/RConn1
  3ph_Dyg/LConn1 -- threephase_vi_measures/RConn1
  3ph_Dyg/LConn2 -- threephase_vi_measures/RConn2
  3ph_Dyg/LConn3 -- threephase_vi_measures/RConn3
  Controlled Voltage Source/LConn1 -- threephase_vi_measures/LConn1
  Controlled Voltage Source1/LConn1 -- threephase_vi_measures/LConn2
  Controlled Voltage Source2/LConn1 -- threephase_vi_measures/LConn3

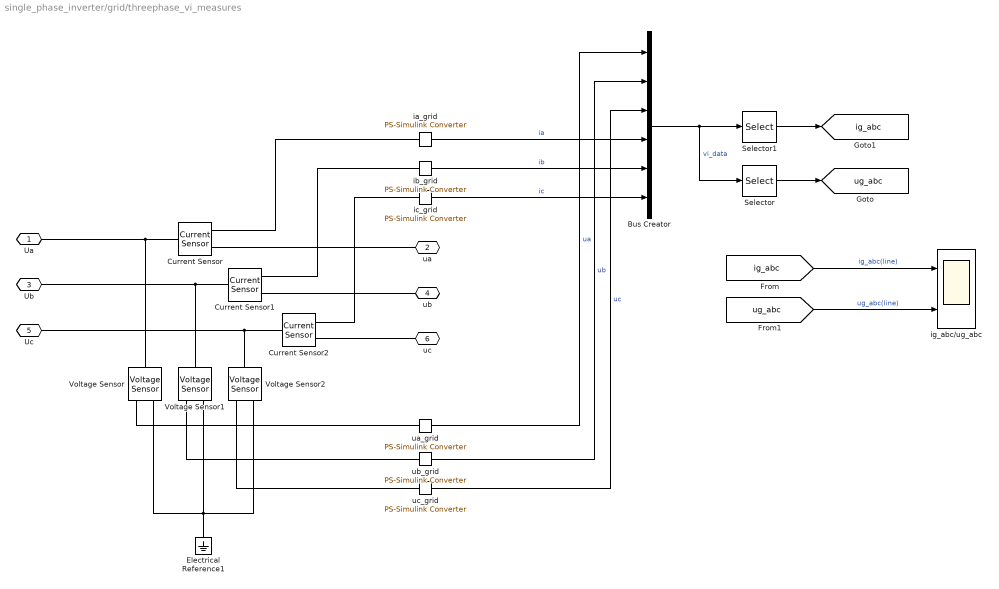
== system single_phase_inverter/grid/threephase_vi_measures ==
  Bus Creator : BusCreator  Inputs=6
  Current Sensor : fl_lib/Electrical/Electrical Sensors/Current Sensor
  Current Sensor1 : fl_lib/Electrical/Electrical Sensors/Current Sensor
  Current Sensor2 : fl_lib/Electrical/Electrical Sensors/Current Sensor
  Electrical Reference1 : fl_lib/Electrical/Electrical Elements/Electrical Reference
  Selector : Selector  InputPortWidth=6  IndexOptions=Index vector (dialog)  Indices=[1 2 3]  OutputSizes=1
  Selector1 : Selector  InputPortWidth=6  IndexOptions=Index vector (dialog)  Indices=[4 5 6]  OutputSizes=1
  Voltage Sensor : fl_lib/Electrical/Electrical Sensors/Voltage Sensor
  Voltage Sensor1 : fl_lib/Electrical/Electrical Sensors/Voltage Sensor
  Voltage Sensor2 : fl_lib/Electrical/Electrical Sensors/Voltage Sensor
  ia_grid : nesl_utility/PS-Simulink Converter  PhysicalDomain=network_engine_domain  SubClassName=ps_output  LeftPortType=input  RightPortType=output  PseudoPeriodic=off  Frequencies=[]  VectorFormat=1-D array  Unit=A  AffineConversion=off
  ib_grid : nesl_utility/PS-Simulink Converter  PhysicalDomain=network_engine_domain  SubClassName=ps_output  LeftPortType=input  RightPortType=output  PseudoPeriodic=off  Frequencies=[]  VectorFormat=1-D array  Unit=A  AffineConversion=off
  ic_grid : nesl_utility/PS-Simulink Converter  PhysicalDomain=network_engine_domain  SubClassName=ps_output  LeftPortType=input  RightPortType=output  PseudoPeriodic=off  Frequencies=[]  VectorFormat=1-D array  Unit=A  AffineConversion=off
  ig_abc/ug_abc : Scope  NumInputPorts=2
      settings: SampleTime=param.glb_time.tc  ActiveDisplayYMinimum=-433.31867245289311  ActiveDisplayYMaximum=433.24358891928017  DataLoggingVariableName=ScopeData2
  ua_grid : nesl_utility/PS-Simulink Converter  PhysicalDomain=network_engine_domain  SubClassName=ps_output  LeftPortType=input  RightPortType=output  PseudoPeriodic=off  Frequencies=[]  VectorFormat=1-D array  Unit=V  AffineConversion=off
  ub_grid : nesl_utility/PS-Simulink Converter  PhysicalDomain=network_engine_domain  SubClassName=ps_output  LeftPortType=input  RightPortType=output  PseudoPeriodic=off  Frequencies=[]  VectorFormat=1-D array  Unit=V  AffineConversion=off
  uc_grid : nesl_utility/PS-Simulink Converter  PhysicalDomain=network_engine_domain  SubClassName=ps_output  LeftPortType=input  RightPortType=output  PseudoPeriodic=off  Frequencies=[]  VectorFormat=1-D array  Unit=V  AffineConversion=off
  Ua : PMIOPort  Side=Left
  ua : PMIOPort  Port=2  Side=Right
  Ub : PMIOPort  Port=3  Side=Left
  ub : PMIOPort  Port=4  Side=Right
  Uc : PMIOPort  Port=5  Side=Left
  uc : PMIOPort  Port=6  Side=Right
  tag scope: ig_abc=global, ug_abc=global
  wires:
  Bus Creator/1 -> Selector1/1, Selector/1  "vi_data"
  Selector/1 -> [ug_abc]
  ib_grid/1 -> Bus Creator/5  "ib"
  ia_grid/1 -> Bus Creator/4  "ia"
  ic_grid/1 -> Bus Creator/6  "ic"
  ua_grid/1 -> Bus Creator/1  "ua"
  ub_grid/1 -> Bus Creator/2  "ub"
  uc_grid/1 -> Bus Creator/3  "uc"
  Selector1/1 -> [ig_abc]
  [ug_abc] -> ig_abc/ug_abc/2  "ug_abc(line)"
  [ig_abc] -> ig_abc/ug_abc/1  "ig_abc(line)"
  connections:
  Current Sensor1/LConn1 -- Ub/RConn1 -- Voltage Sensor1/LConn1
  Electrical Reference1/LConn1 -- Voltage Sensor/RConn2 -- Voltage Sensor2/RConn2 -- Voltage Sensor1/RConn2
  Voltage Sensor/RConn1 -- ua_grid/LConn1
  Current Sensor/RConn2 -- ua/RConn1
  Voltage Sensor1/RConn1 -- ub_grid/LConn1
  Voltage Sensor2/LConn1 -- Current Sensor2/LConn1 -- Uc/RConn1
  Current Sensor/LConn1 -- Ua/RConn1 -- Voltage Sensor/LConn1
  Current Sensor1/RConn2 -- ub/RConn1
  Voltage Sensor2/RConn1 -- uc_grid/LConn1
  ib_grid/LConn1 -- Current Sensor1/RConn1
  ia_grid/LConn1 -- Current Sensor/RConn1
  ic_grid/LConn1 -- Current Sensor2/RConn1
  Current Sensor2/RConn2 -- uc/RConn1

== system single_phase_inverter/rectifier/H5_filter ==
  Capacitor : fl_lib/Electrical/Electrical Elements/Capacitor  c=C5 F  r=1e-6 Ohm  g=0 1/Ohm  i_specify=off  i_priority=None  i=0 A  i_nominal_specify=off  i_nominal_value=1  i_nominal_unit=A  v_specify=off  v_priority=None  v=0 V  v_nominal_specify=off  v_nominal_value=1  v_nominal_unit=V  vc_specify=off  vc_priority=High  vc=0 V  vc_nominal_specify=off  vc_nominal_value=1  vc_nominal_unit=V
  Capacitor1 : fl_lib/Electrical/Electrical Elements/Capacitor  c=C5 F  r=1e-6 Ohm  g=0 1/Ohm  i_specify=off  i_priority=None  i=0 A  i_nominal_specify=off  i_nominal_value=1  i_nominal_unit=A  v_specify=off  v_priority=None  v=0 V  v_nominal_specify=off  v_nominal_value=1  v_nominal_unit=V  vc_specify=off  vc_priority=High  vc=0 V  vc_nominal_specify=off  vc_nominal_value=1  vc_nominal_unit=V
  Capacitor2 : fl_lib/Electrical/Electrical Elements/Capacitor  c=C5 F  r=1e-6 Ohm  g=0 1/Ohm  i_specify=off  i_priority=None  i=0 A  i_nominal_specify=off  i_nominal_value=1  i_nominal_unit=A  v_specify=off  v_priority=None  v=0 V  v_nominal_specify=off  v_nominal_value=1  v_nominal_unit=V  vc_specify=off  vc_priority=High  vc=0 V  vc_nominal_specify=off  vc_nominal_value=1  vc_nominal_unit=V
  Inductor5 : fl_lib/Electrical/Electrical Elements/Inductor  l=L5 H  r=0 Ohm  g=1e-9 1/Ohm  i_specify=off  i_priority=None  i=0 A  i_nominal_specify=off  i_nominal_value=1  i_nominal_unit=A  v_specify=off  v_priority=None  v=0 V  v_nominal_specify=off  v_nominal_value=1  v_nominal_unit=V  i_L_specify=off  i_L_priority=High  i_L=0 A  i_L_nominal_specify=off  i_L_nominal_value=1  i_L_nominal_unit=A
  Inductor6 : fl_lib/Electrical/Electrical Elements/Inductor  l=L5 H  r=0 Ohm  g=1e-9 1/Ohm  i_specify=off  i_priority=None  i=0 A  i_nominal_specify=off  i_nominal_value=1  i_nominal_unit=A  v_specify=off  v_priority=None  v=0 V  v_nominal_specify=off  v_nominal_value=1  v_nominal_unit=V  i_L_specify=off  i_L_priority=High  i_L=0 A  i_L_nominal_specify=off  i_L_nominal_value=1  i_L_nominal_unit=A
  Inductor7 : fl_lib/Electrical/Electrical Elements/Inductor  l=L5 H  r=0 Ohm  g=1e-9 1/Ohm  i_specify=off  i_priority=None  i=0 A  i_nominal_specify=off  i_nominal_value=1  i_nominal_unit=A  v_specify=off  v_priority=None  v=0 V  v_nominal_specify=off  v_nominal_value=1  v_nominal_unit=V  i_L_specify=off  i_L_priority=High  i_L=0 A  i_L_nominal_specify=off  i_L_nominal_value=1  i_L_nominal_unit=A
  w : PMIOPort  Side=Left
  v : PMIOPort  Port=2  Side=Left
  u : PMIOPort  Port=3  Side=Left
  connections:
  Capacitor2/LConn1 -- Inductor7/RConn1
  Inductor5/LConn1 -- w/RConn1
  Capacitor/RConn1 -- Capacitor2/RConn1 -- Capacitor1/RConn1
  Capacitor/LConn1 -- Inductor5/RConn1
  Capacitor1/LConn1 -- Inductor6/RConn1
  Inductor7/LConn1 -- u/RConn1
  Inductor6/LConn1 -- v/RConn1

== system single_phase_inverter/rectifier/H7_filter ==
  Capacitor1 : fl_lib/Electrical/Electrical Elements/Capacitor  c=C7 F  r=1e-6 Ohm  g=0 1/Ohm  i_specify=off  i_priority=None  i=0 A  i_nominal_specify=off  i_nominal_value=1  i_nominal_unit=A  v_specify=off  v_priority=None  v=0 V  v_nominal_specify=off  v_nominal_value=1  v_nominal_unit=V  vc_specify=off  vc_priority=High  vc=0 V  vc_nominal_specify=off  vc_nominal_value=1  vc_nominal_unit=V
  Capacitor2 : fl_lib/Electrical/Electrical Elements/Capacitor  c=C7 F  r=1e-6 Ohm  g=0 1/Ohm  i_specify=off  i_priority=None  i=0 A  i_nominal_specify=off  i_nominal_value=1  i_nominal_unit=A  v_specify=off  v_priority=None  v=0 V  v_nominal_specify=off  v_nominal_value=1  v_nominal_unit=V  vc_specify=off  vc_priority=High  vc=0 V  vc_nominal_specify=off  vc_nominal_value=1  vc_nominal_unit=V
  Capacitor3 : fl_lib/Electrical/Electrical Elements/Capacitor  c=C7 F  r=1e-6 Ohm  g=0 1/Ohm  i_specify=off  i_priority=None  i=0 A  i_nominal_specify=off  i_nominal_value=1  i_nominal_unit=A  v_specify=off  v_priority=None  v=0 V  v_nominal_specify=off  v_nominal_value=1  v_nominal_unit=V  vc_specify=off  vc_priority=High  vc=0 V  vc_nominal_specify=off  vc_nominal_value=1  vc_nominal_unit=V
  Inductor1 : fl_lib/Electrical/Electrical Elements/Inductor  l=L7 H  r=0 Ohm  g=1e-9 1/Ohm  i_specify=off  i_priority=None  i=0 A  i_nominal_specify=off  i_nominal_value=1  i_nominal_unit=A  v_specify=off  v_priority=None  v=0 V  v_nominal_specify=off  v_nominal_value=1  v_nominal_unit=V  i_L_specify=off  i_L_priority=High  i_L=0 A  i_L_nominal_specify=off  i_L_nominal_value=1  i_L_nominal_unit=A
  Inductor2 : fl_lib/Electrical/Electrical Elements/Inductor  l=L7 H  r=0 Ohm  g=1e-9 1/Ohm  i_specify=off  i_priority=None  i=0 A  i_nominal_specify=off  i_nominal_value=1  i_nominal_unit=A  v_specify=off  v_priority=None  v=0 V  v_nominal_specify=off  v_nominal_value=1  v_nominal_unit=V  i_L_specify=off  i_L_priority=High  i_L=0 A  i_L_nominal_specify=off  i_L_nominal_value=1  i_L_nominal_unit=A
  Inductor7 : fl_lib/Electrical/Electrical Elements/Inductor  l=L7 H  r=0 Ohm  g=1e-9 1/Ohm  i_specify=off  i_priority=None  i=0 A  i_nominal_specify=off  i_nominal_value=1  i_nominal_unit=A  v_specify=off  v_priority=None  v=0 V  v_nominal_specify=off  v_nominal_value=1  v_nominal_unit=V  i_L_specify=off  i_L_priority=High  i_L=0 A  i_L_nominal_specify=off  i_L_nominal_value=1  i_L_nominal_unit=A
  w : PMIOPort  Side=Left
  v : PMIOPort  Port=2  Side=Left
  u : PMIOPort  Port=3  Side=Left
  connections:
  Inductor1/LConn1 -- v/RConn1
  Inductor7/LConn1 -- u/RConn1
  Capacitor1/LConn1 -- Inductor1/RConn1
  Capacitor3/LConn1 -- Inductor2/RConn1
  Capacitor2/RConn1 -- Capacitor3/RConn1 -- Capacitor1/RConn1
  Inductor2/LConn1 -- w/RConn1
  Capacitor2/LConn1 -- Inductor7/RConn1

== system single_phase_inverter/single_phase_inverter/single phase inverter ==
  gate_commands : Inport
  full_bridge_ideal_switch_based : Subsystem
  full_bridge_mosfet_based_with_thermal_model : Subsystem  Commented=on
  uac_out(+) : PMIOPort  Side=Left
  uac_out(-) : PMIOPort  Port=2  Side=Left
  udc(+) : PMIOPort  Port=3  Side=Right
  udc(-) : PMIOPort  Port=4  Side=Right
  wires:
  gate_commands/1 -> full_bridge_ideal_switch_based/1(gate_commands), full_bridge_mosfet_based_with_thermal_model/1(gate_commands)
  connections:
  full_bridge_mosfet_based_with_thermal_model/LConn1 -- full_bridge_ideal_switch_based/LConn1 -- udc(+)/RConn1
  full_bridge_mosfet_based_with_thermal_model/RConn1 -- uac_out(+)/RConn1 -- full_bridge_ideal_switch_based/RConn1
  full_bridge_mosfet_based_with_thermal_model/LConn2 -- full_bridge_ideal_switch_based/LConn2 -- udc(-)/RConn1
  full_bridge_mosfet_based_with_thermal_model/RConn2 -- uac_out(-)/RConn1 -- full_bridge_ideal_switch_based/RConn2

== system single_phase_inverter/single_phase_inverter/single phase inverter control ==
  Terminator : Terminator
  acquisition_and_scaling_current : Subsystem  Commented=on
  acquisition_and_scaling_current_with_white_noise : Subsystem
  acquisition_and_scaling_dc_voltage : Subsystem
  acquisition_and_scaling_grid_voltage_ac : Subsystem
  acquisition_and_scaling_voltage : Subsystem
  inverter_current_output_pu_reference : Subsystem
  pwm modulator : Subsystem
  single_phase_inverter_ctrl : Subsystem
  gate_cmds : Outport
  wires:
  [inverter_current_output] -> acquisition_and_scaling_current_with_white_noise/1(in)
  pwm modulator/1(gate_cmds) -> gate_cmds/1
  [TRGO_INV_1] -> single_phase_inverter_ctrl/Trigger
  [inverter_voltage_output] -> acquisition_and_scaling_voltage/1(in)
  single_phase_inverter_ctrl/1(u_ctrl_out) -> pwm modulator/1(vout)
  acquisition_and_scaling_current_with_white_noise/1(out) -> single_phase_inverter_ctrl/2(inverter_current_output_pu)  "inverter_current_output_pu"
  acquisition_and_scaling_voltage/1(out) -> single_phase_inverter_ctrl/1(inverter_voltage_output_pu)  "inverter_voltage_output_pu"
  inverter_current_output_pu_reference/1(inverter_current_output_pu_reference) -> single_phase_inverter_ctrl/3(inverter_current output_pu_reference)  "inverter_current_output_pu_reference"
  [dclink_voltage] -> acquisition_and_scaling_dc_voltage/1(in)
  acquisition_and_scaling_dc_voltage/1(out) -> single_phase_inverter_ctrl/4(dclink_voltage_pu)  "dclink_voltage_pu"
  [time_inv_module_1] -> single_phase_inverter_ctrl/5(local_time)
  [ug_abc] -> acquisition_and_scaling_grid_voltage_ac/1(in)
  acquisition_and_scaling_grid_voltage_ac/1(out) -> single_phase_inverter_ctrl/6(ugrid_pu)  "ug_abc"
  single_phase_inverter_ctrl/2(m) -> Terminator/1

== system single_phase_inverter/grid/grid_emulator/3ph_Dyg ==
  Electrical Reference1 : fl_lib/Electrical/Electrical Elements/Electrical Reference
  ph1 : single_phase_transformer_lib/single phase transformer  Lm=param.grid.emu.trafo.Lm1 H  n1=param.grid.emu.trafo.n1  n2=param.grid.emu.trafo.n2  Rd1=param.grid.emu.trafo.Rd1 Ohm  Rd2=param.grid.emu.trafo.Rd2 Ohm  Ld1=param.grid.emu.trafo.Ld1 H  Ld2=param.grid.emu.trafo.Ld2 H  Rfe=param.grid.emu.trafo.Rfe1 Ohm  phi_specify=off  phi_priority=None  phi=0 V*s  phi_nominal_specify=off  phi_nominal_value=1  phi_nominal_unit=V*s  i1_specify=off  i1_priority=None  i1=0 A  i1_nominal_specify=off  i1_nominal_value=1  i1_nominal_unit=A  i2_specify=off  i2_priority=None  i2=0 A  i2_nominal_specify=off  i2_nominal_value=1  i2_nominal_unit=A  ife_specify=off  ife_priority=None  ife=0 A  ife_nominal_specify=off  ife_nominal_value=1  ife_nominal_unit=A  u1_specify=off  u1_priority=None  u1=0 V  u1_nominal_specify=off  u1_nominal_value=1  u1_nominal_unit=V  u2_specify=off  u2_priority=None  u2=0 V  u2_nominal_specify=off  u2_nominal_value=1  u2_nominal_unit=V
  ph2 : single_phase_transformer_lib/single phase transformer  Lm=param.grid.emu.trafo.Lm1 H  n1=param.grid.emu.trafo.n1  n2=param.grid.emu.trafo.n2  Rd1=param.grid.emu.trafo.Rd1 Ohm  Rd2=param.grid.emu.trafo.Rd2 Ohm  Ld1=param.grid.emu.trafo.Ld1 H  Ld2=param.grid.emu.trafo.Ld2 H  Rfe=param.grid.emu.trafo.Rfe1 Ohm  phi_specify=off  phi_priority=None  phi=0 V*s  phi_nominal_specify=off  phi_nominal_value=1  phi_nominal_unit=V*s  i1_specify=off  i1_priority=None  i1=0 A  i1_nominal_specify=off  i1_nominal_value=1  i1_nominal_unit=A  i2_specify=off  i2_priority=None  i2=0 A  i2_nominal_specify=off  i2_nominal_value=1  i2_nominal_unit=A  ife_specify=off  ife_priority=None  ife=0 A  ife_nominal_specify=off  ife_nominal_value=1  ife_nominal_unit=A  u1_specify=off  u1_priority=None  u1=0 V  u1_nominal_specify=off  u1_nominal_value=1  u1_nominal_unit=V  u2_specify=off  u2_priority=None  u2=0 V  u2_nominal_specify=off  u2_nominal_value=1  u2_nominal_unit=V
  ph3 : single_phase_transformer_lib/single phase transformer  Lm=param.grid.emu.trafo.Lm1 H  n1=param.grid.emu.trafo.n1  n2=param.grid.emu.trafo.n2  Rd1=param.grid.emu.trafo.Rd1 Ohm  Rd2=param.grid.emu.trafo.Rd2 Ohm  Ld1=param.grid.emu.trafo.Ld1 H  Ld2=param.grid.emu.trafo.Ld2 H  Rfe=param.grid.emu.trafo.Rfe1 Ohm  phi_specify=off  phi_priority=None  phi=0 V*s  phi_nominal_specify=off  phi_nominal_value=1  phi_nominal_unit=V*s  i1_specify=off  i1_priority=None  i1=0 A  i1_nominal_specify=off  i1_nominal_value=1  i1_nominal_unit=A  i2_specify=off  i2_priority=None  i2=0 A  i2_nominal_specify=off  i2_nominal_value=1  i2_nominal_unit=A  ife_specify=off  ife_priority=None  ife=0 A  ife_nominal_specify=off  ife_nominal_value=1  ife_nominal_unit=A  u1_specify=off  u1_priority=None  u1=0 V  u1_nominal_specify=off  u1_nominal_value=1  u1_nominal_unit=V  u2_specify=off  u2_priority=None  u2=0 V  u2_nominal_specify=off  u2_nominal_value=1  u2_nominal_unit=V
  ua : PMIOPort  Side=Right
  ub : PMIOPort  Port=2  Side=Right
  uc : PMIOPort  Port=3  Side=Right
  Ua : PMIOPort  Port=4  Side=Left
  Ub : PMIOPort  Port=5  Side=Left
  Uc : PMIOPort  Port=6  Side=Left
  connections:
  Electrical Reference1/LConn1 -- ph3/RConn2 -- ph2/RConn2 -- ph1/RConn2
  ph3/RConn1 -- uc/RConn1
  ph1/LConn1 -- ph3/LConn2 -- Ua/RConn1
  ph1/RConn1 -- ua/RConn1
  ph2/RConn1 -- ub/RConn1
  ph1/LConn2 -- ph2/LConn1 -- Ub/RConn1
  Uc/RConn1 -- ph3/LConn1 -- ph2/LConn2
